simulink model "torque_vectoring_sim"  (R2022a)
settings: Solver=FixedStepAuto  StartTime=0.0  StopTime=5  FixedStep=0.01  RelTol=1e-3
undefined symbols (not defined in the file): DiscIntNeverNeededParam
libraries: simulink_extras x2, simulink x1
(part 2 of 2)

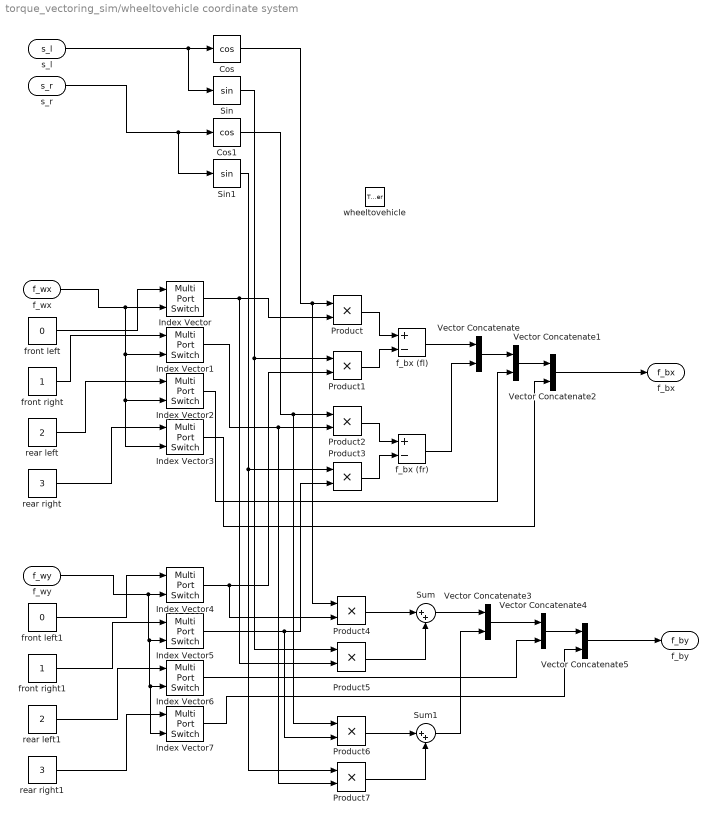
== system torque_vectoring_sim/wheeltovehicle coordinate system ==
  wheeltovehicle : TriggerPort  TriggerType=function-call  IsSimulinkFunction=on  FunctionName=wheeltovehicle  FunctionVisibility=scoped  VariantControl=(inherit)
  Cos : Trigonometry  Operator=cos
  Cos1 : Trigonometry  Operator=cos
  Index Vector{,1..7} (8 alike) : MultiPortSwitch  DataPortOrder=Zero-based contiguous  Inputs=1  zeroidx=on  SaturateOnIntegerOverflow=off  InputSameDT=off
  Product{,1..7} (8 alike) : Product
  Sin : Trigonometry
  Sin1 : Trigonometry
  Sum : Sum  Inputs=|++
  Sum1 : Sum  Inputs=|++
  Vector Concatenate{,1..5} (6 alike) : Concatenate
  f_bx (fl) : Sum  Inputs=+-
  f_bx (fr) : Sum  Inputs=+-
  front left : Constant  Value=0
  front left1 : Constant  Value=0
  front right : Constant
  front right1 : Constant
  rear left : Constant  Value=2
  rear left1 : Constant  Value=2
  rear right : Constant  Value=3
  rear right1 : Constant  Value=3
  f_wx : ArgIn  DisableCoverage=on  PortDimensions=4  ArgumentName=f_wx
  f_wy : ArgIn  Port=2  PortDimensions=4  ArgumentName=f_wy
  s_l : ArgIn  Port=3  ArgumentName=s_l
  s_r : ArgIn  Port=4  ArgumentName=s_r
  f_bx : ArgOut  DisableCoverage=on  PortDimensions=4  ArgumentName=f_bx
  f_by : ArgOut  Port=2  PortDimensions=4  ArgumentName=f_by
  wires:
  f_wx/1 -> Index Vector3/2, Index Vector2/2, Index Vector1/2, Index Vector/2
  s_l/1 -> Sin/1, Cos/1
  s_r/1 -> Sin1/1, Cos1/1
  Index Vector/1 -> Product5/2, Product/2
  Index Vector4/1 -> Product4/2, Product1/2
  Sin/1 -> Product5/1, Product1/1
  Product/1 -> f_bx (fl)/1
  Product1/1 -> f_bx (fl)/2
  Index Vector1/1 -> Product7/2, Product2/2
  Cos1/1 -> Product6/1, Product2/1
  Sin1/1 -> Product7/1, Product3/1
  Index Vector5/1 -> Product6/2, Product3/2
  Product3/1 -> f_bx (fr)/2
  Product2/1 -> f_bx (fr)/1
  Index Vector2/1 -> Vector Concatenate1/2
  Index Vector3/1 -> Vector Concatenate2/2
  Product4/1 -> Sum/1
  Product5/1 -> Sum/2
  Product6/1 -> Sum1/1
  Product7/1 -> Sum1/2
  Cos/1 -> Product4/1, Product/1
  Index Vector6/1 -> Vector Concatenate4/2
  Index Vector7/1 -> Vector Concatenate5/2
  f_bx (fl)/1 -> Vector Concatenate/1
  f_bx (fr)/1 -> Vector Concatenate/2
  Vector Concatenate/1 -> Vector Concatenate1/1
  Vector Concatenate1/1 -> Vector Concatenate2/1
  Vector Concatenate2/1 -> f_bx/1
  Sum/1 -> Vector Concatenate3/1
  Sum1/1 -> Vector Concatenate3/2
  Vector Concatenate3/1 -> Vector Concatenate4/1
  Vector Concatenate4/1 -> Vector Concatenate5/1
  Vector Concatenate5/1 -> f_by/1
  rear right/1 -> Index Vector3/1
  rear left/1 -> Index Vector2/1
  front right/1 -> Index Vector1/1
  front left/1 -> Index Vector/1
  f_wy/1 -> Index Vector7/2, Index Vector6/2, Index Vector5/2, Index Vector4/2
  front left1/1 -> Index Vector4/1
  front right1/1 -> Index Vector5/1
  rear left1/1 -> Index Vector6/1
  rear right1/1 -> Index Vector7/1

== system torque_vectoring_sim/Desired Yaw1/If Action Subsystem ==
  In1 : Inport
  Action Port : ActionPort  ActionPortLabel=else
  Out1 : Outport
  wires:
  In1/1 -> Out1/1

== system torque_vectoring_sim/Desired Yaw1/If Action Subsystem1 ==
  In1 : Inport
  Action Port : ActionPort  ActionPortLabel=if(u2 < u1)
  Out1 : Outport
  wires:
  In1/1 -> Out1/1

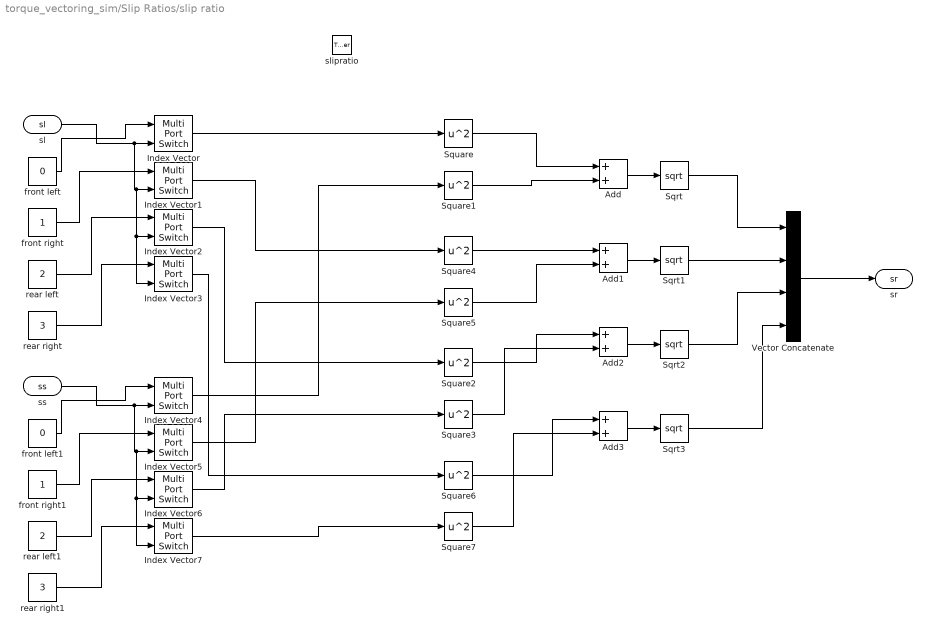
== system torque_vectoring_sim/Slip Ratios/slip ratio ==
  slipratio : TriggerPort  TriggerType=function-call  IsSimulinkFunction=on  FunctionName=slipratio  FunctionVisibility=scoped  VariantControl=(inherit)
  Add{,1..3} (4 alike) : Sum
  Index Vector{,1..7} (8 alike) : MultiPortSwitch  DataPortOrder=Zero-based contiguous  Inputs=1  zeroidx=on  SaturateOnIntegerOverflow=off  InputSameDT=off
  Sqrt{,1..3} (4 alike) : Sqrt
  Square{,1..7} (8 alike) : Math  Operator=square
  Vector Concatenate : Concatenate  NumInputs=4
  front left : Constant  Value=0
  front left1 : Constant  Value=0
  front right : Constant
  front right1 : Constant
  rear left : Constant  Value=2
  rear left1 : Constant  Value=2
  rear right : Constant  Value=3
  rear right1 : Constant  Value=3
  sl : ArgIn  DisableCoverage=on  PortDimensions=4  ArgumentName=sl
  ss : ArgIn  Port=2  PortDimensions=4  ArgumentName=ss
  sr : ArgOut  DisableCoverage=on  PortDimensions=4  ArgumentName=sr
  wires:
  rear right/1 -> Index Vector3/1
  sl/1 -> Index Vector3/2, Index Vector2/2, Index Vector1/2, Index Vector/2
  front left/1 -> Index Vector/1
  front right/1 -> Index Vector1/1
  rear left/1 -> Index Vector2/1
  rear right1/1 -> Index Vector7/1
  ss/1 -> Index Vector7/2, Index Vector6/2, Index Vector5/2, Index Vector4/2
  front left1/1 -> Index Vector4/1
  front right1/1 -> Index Vector5/1
  rear left1/1 -> Index Vector6/1
  Add1/1 -> Sqrt1/1
  Add2/1 -> Sqrt2/1
  Add/1 -> Sqrt/1
  Add3/1 -> Sqrt3/1
  Square/1 -> Add/1
  Square1/1 -> Add/2
  Square4/1 -> Add1/1
  Square5/1 -> Add1/2
  Square2/1 -> Add2/1
  Square3/1 -> Add2/2
  Square6/1 -> Add3/1
  Square7/1 -> Add3/2
  Index Vector/1 -> Square/1
  Index Vector4/1 -> Square1/1
  Index Vector1/1 -> Square4/1
  Index Vector5/1 -> Square5/1
  Index Vector2/1 -> Square2/1
  Index Vector6/1 -> Square3/1
  Index Vector7/1 -> Square7/1
  Index Vector3/1 -> Square6/1
  Sqrt/1 -> Vector Concatenate/1
  Sqrt1/1 -> Vector Concatenate/2
  Sqrt2/1 -> Vector Concatenate/3
  Sqrt3/1 -> Vector Concatenate/4
  Vector Concatenate/1 -> sr/1

== system torque_vectoring_sim/tiremodelburckhardt/u_r Burkhardt equation ==
  burk : TriggerPort  TriggerType=function-call  IsSimulinkFunction=on  FunctionName=burk  FunctionVisibility=scoped  VariantControl=(inherit)
  C1 : Constant  Value=1.2801
  C2 : Constant  Value=23.99
  C3 : Constant  Value=0.52
  Constant : Constant
  Eulers Number : Constant  Value=exp(1)  OutDataTypeStr=Inherit: Inherit via back propagation
  Gain : Gain  Gain=-1
  Power : Math  Operator=pow  OutputSignalType=real
  Product : Product
  Product1 : Product
  Product2 : Product
  Subtract : Sum  Inputs=+-
  Subtract1 : Sum  Inputs=+-
  sr : ArgIn  DisableCoverage=on  ArgumentName=sr
  ur : ArgOut  DisableCoverage=on  ArgumentName=ur
  wires:
  Constant/1 -> Subtract/1
  Eulers Number/1 -> Power/1
  Product1/1 -> Power/2
  Power/1 -> Subtract/2
  Gain/1 -> Product1/2
  C2/1 -> Gain/1
  C1/1 -> Product/1
  Subtract/1 -> Product/2
  Product/1 -> Subtract1/1
  sr/1 -> Product2/1, Product1/1
  C3/1 -> Product2/2
  Product2/1 -> Subtract1/2
  Subtract1/1 -> ur/1

== matlab function torque_vectoring_sim/Slip Ratios/Longitudinal Slip ==
  data: w input; r input; a input; v input; fl output; fr output; rl output; rr output
function [fl,fr,rl,rr] = longSlip(w,r,a,v)
    fl = (w(1) * r * cos(a(1)) - v(1))/(w(1) * r * cos(a(1)));
    fr = (w(2) * r * cos(a(2)) - v(2))/(w(2) * r * cos(a(2)));
    rl = (w(3) * r * cos(a(3)) - v(3))/(w(3) * r * cos(a(3)));
    rr = (w(4) * r * cos(a(4)) - v(4))/(w(4) * r * cos(a(4)));
end

== matlab function torque_vectoring_sim/Slip Ratios/Lateral Slip ==
  data: a input; fl output; fr output; rl output; rr output
function [fl,fr,rl,rr] = latSlip(a)
    fl = tan(a(1));
    fr = tan(a(2));
    rl = tan(a(3));
    rr = tan(a(4));
end

== matlab function torque_vectoring_sim/Rolling Force/F_yroll ==
  data: c input; fl output; f input; w input; sl input; fr output; sr input
function [fl,fr] = fcn(c,f,w,sl,sr)
    fl = c*f(1)*sign(w(1))*sin(sl);
    fr = c*f(2)*sign(w(2))*sin(sr);
end

== matlab function torque_vectoring_sim/Rolling Force/F_xroll ==
  data: c input; fl output; f input; w input; sl input; fr output; rl output; rr output; sr input
function [fl,fr,rl,rr] = fcn(c,f,w,sl,sr)
    fl = c * f(1) * sign(w(1)) * cos(sl);
    fr = c * f(2) * sign(w(2)) * cos(sr);
    rl = c * f(3) * sign(w(3));
    rr = c * f(4) * sign(w(4));
end
